simulink model "TB02_StageB_HBridge"  (R2025a)
settings: Solver=FixedStepDiscrete  StartTime=0  StopTime=TB.t_end  FixedStep=TB.dt  RelTol=1e-3
InitFcn:
  | % 모델과 같은 폴더의 초기화 스크립트를 실행해 P(설계 파라미터)와 TB(시험 조건)를 만든다.
  | run(fullfile(fileparts(get_param(bdroot, 'FileName')), 'TB02_init.m'));
values from neighbouring files (symbols this model uses):
  TB = struct()    [TB02_init.m]
libraries: fl_lib x20, nesl_utility x8
settings Model: Creator=hj000  LastModifiedBy=hj000
settings DataIOCC: SaveOutput=off  SignalLogging=off  SaveTime=off

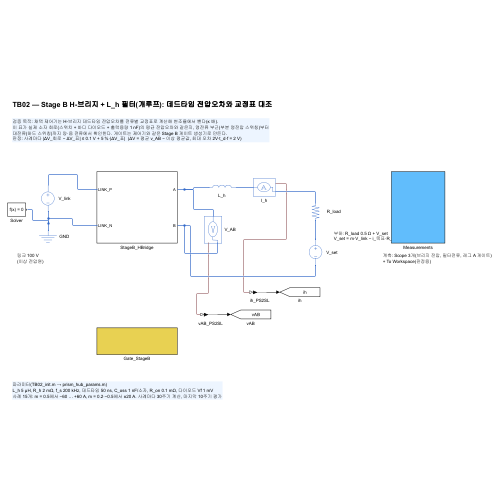
[thumbnail: Simulink's stored preview of the top-level diagram]
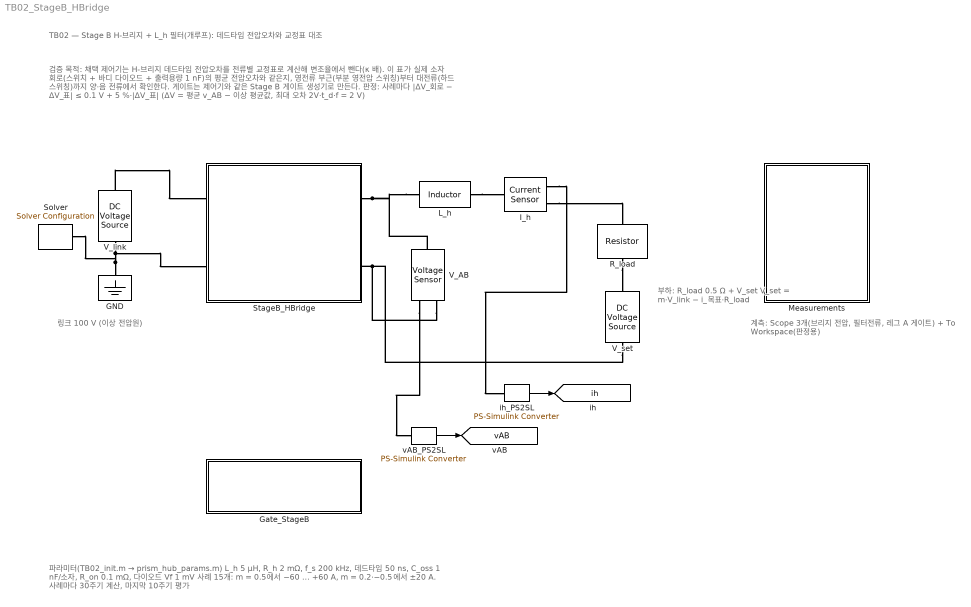
== system TB02_StageB_HBridge ==
  note: TB02 — Stage B H-브리지 + L_h 필터(개루프): 데드타임 전압오차와 교정표 대조
  note: 검증 목적: 채택 제어기는 H-브리지 데드타임 전압오차를 전류별 교정표로 계산해 변조율에서 뺀다(κ 배).
      | 이 표가 실제 소자 회로(스위치 + 바디 다이오드 + 출력용량 1 nF)의 평균 전압오차와 같은지, 영전류 부근(부분 영전압 스위칭)부터
      | 대전류(하드 스위칭)까지 양·음 전류에서 확인한다. 게이트는 제어기와 같은 Stage B 게이트 생성기로 만든다.
      | 판정: 사례마다 |ΔV_회로 − ΔV_표| ≤ 0.1 V + 5 %·|ΔV_표|  (ΔV = 평균 v_AB − 이상 평균값, 최대 오차 2V·t_d·f = 2 V)
  note: 링크 100 V
      | (이상 전압원)
  note: 부하: R_load 0.5 Ω + V_set
      | V_set = m·V_link − i_목표·R_load
  note: 계측: Scope 3개(브리지 전압, 필터전류, 레그 A 게이트)
      | + To Workspace(판정용)
  note: 파라미터(TB02_init.m → prism_hub_params.m)
      | L_h 5 µH, R_h 2 mΩ, f_s 200 kHz, 데드타임 50 ns, C_oss 1 nF/소자, R_on 0.1 mΩ, 다이오드 Vf 1 mV
      | 사례 15개: m = 0.5에서 −60 … +60 A, m = 0.2·−0.5에서 ±20 A. 사례마다 30주기 계산, 마지막 10주기 평가
  GND : fl_lib/Electrical/Electrical Elements/Electrical Reference
  Gate_StageB : Subsystem
  I_h : fl_lib/Electrical/Electrical Sensors/Current Sensor
  L_h : fl_lib/Electrical/Electrical Elements/Inductor  l=TB.B.Lh H  r=TB.B.Rh Ohm  g=1e-9 1/Ohm  i_specify=off  i_priority=None  i=0 A  i_nominal_specify=off  i_nominal_value=1  i_nominal_unit=A  v_specify=off  v_priority=None  v=0 V  v_nominal_specify=off  v_nominal_value=1  v_nominal_unit=V  i_L_specify=on  i_L_priority=High  i_L=TB.i0 A  i_L_nominal_specify=off  i_L_nominal_value=1  i_L_nominal_unit=A
  Measurements : Subsystem
  R_load : fl_lib/Electrical/Electrical Elements/Resistor  R=TB.Rload Ohm  i_specify=off  i_priority=None  i=0 A  i_nominal_specify=off  i_nominal_value=1  i_nominal_unit=A  v_specify=off  v_priority=None  v=0 V  v_nominal_specify=off  v_nominal_value=1  v_nominal_unit=V
  Solver : nesl_utility/Solver Configuration  PhysicalDomain=network_engine_domain  SubClassName=solver  LeftPortType=input  RightPortType=generic  Tones=[]  Harmonics=[]  SimulateNoise=off  Profile=off  UseLocalSampling=off  EnableSwitchedLinearOptims=on  FrequencyDomain=off  UseCCode=off  RelTol=0.001  AbsTol=0.001  MinStep=1e-09  ToWorkspace=off  RevertToSquareIcSolve=off  NumHomotopyIterations=100  PhasorMode=off  PhasorModeNumHarmonics=1  ConsistencySolver=NEWTON_XTOL_AFTER_FTOL  IndexReductionMethod=DerivativeReplacement  DoDC=off  ResidualTolerance=1e-9  ConsistencyTolSource=GLOBAL  ConsistencyAbsTol=0.001  ConsistencyRelTol=0.001  ConsistencyTolFactor=0.001  UseLocalSolver=on  LocalSolverChoice=NE_BACKWARD_EULER_ADVANCER  ResolveIndetEquations=on  FunctionEvalNumThread=1  LocalSolverSampleTime=TB.dt  DoFixedCost=off  MaxNonlinIter=3  MaxModeIter=2  ComputeImpulses=off  ImpulseIterations=2  LinearAlgebra=auto  LinearAlgebraNumThread=0  EquationFormulation=NE_TIME_EF  DelaysMemoryBudget=1024  AutomaticFiltering=on  FilteringTimeConstant=0.001  PartitionStorageMethod=AS_NEEDED  PartitionMemoryBudget=1024  PartitionMethod=ROBUST  MultibodyUseLocalSolver=off  MultibodyLocalSolverChoice=ODE1  MultibodyLocalSolverSampleTime=0.001
  StageB_HBridge : Subsystem
  V_AB : fl_lib/Electrical/Electrical Sensors/Voltage Sensor
  V_link : fl_lib/Electrical/Electrical Sources/DC Voltage Source  v0=TB.Vlink V
  V_set : fl_lib/Electrical/Electrical Sources/DC Voltage Source  v0=TB.Vset V
  ih_PS2SL : nesl_utility/PS-Simulink Converter  PhysicalDomain=network_engine_domain  SubClassName=ps_output  LeftPortType=input  RightPortType=output  PseudoPeriodic=off  Frequencies=[]  VectorFormat=inherit  Unit=inherit  AffineConversion=off
  vAB_PS2SL : nesl_utility/PS-Simulink Converter  PhysicalDomain=network_engine_domain  SubClassName=ps_output  LeftPortType=input  RightPortType=output  PseudoPeriodic=off  Frequencies=[]  VectorFormat=inherit  Unit=inherit  AffineConversion=off
  tag scope: ih=global, vAB=global
  wires:
  ih_PS2SL/1 -> [ih]
  vAB_PS2SL/1 -> [vAB]
  connections:
  GND/LConn1 -- Solver/RConn1 -- V_link/RConn1 -- StageB_HBridge/LConn2
  V_link/LConn1 -- StageB_HBridge/LConn1
  L_h/LConn1 -- StageB_HBridge/RConn1 -- V_AB/LConn1
  L_h/RConn1 -- I_h/LConn1
  I_h/RConn2 -- R_load/LConn1
  R_load/RConn1 -- V_set/LConn1
  StageB_HBridge/RConn2 -- V_set/RConn1 -- V_AB/RConn2
  I_h/RConn1 -- ih_PS2SL/LConn1
  V_AB/RConn1 -- vAB_PS2SL/LConn1

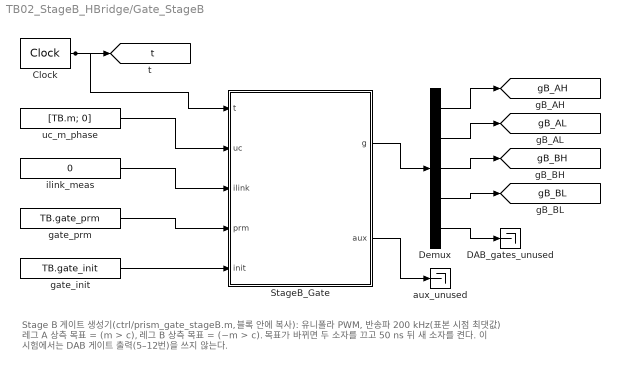
== system TB02_StageB_HBridge/Gate_StageB ==
  note: Stage B 게이트 생성기(ctrl/prism_gate_stageB.m, 블록 안에 복사): 유니폴라 PWM, 반송파 200 kHz(표본 시점 최댓값)
      | 레그 A 상측 목표 = (m > c), 레그 B 상측 목표 = (−m > c). 목표가 바뀌면 두 소자를 끄고 50 ns 뒤 새 소자를 켠다.
      | 이 시험에서는 DAB 게이트 출력(5–12번)을 쓰지 않는다.
  Clock : DigitalClock  SampleTime=TB.dt
  DAB_gates_unused : Terminator
  Demux : Demux  Outputs=[1 1 1 1 8]
  StageB_Gate : MATLAB Function  TreatAsAtomicUnit=on
  aux_unused : Terminator
  gate_init : Constant  Value=TB.gate_init
  gate_prm : Constant  Value=TB.gate_prm
  ilink_meas : Constant  Value=0
  uc_m_phase : Constant  Value=[TB.m; 0]
  tag scope: gB_AH=global, gB_AL=global, gB_BH=global, gB_BL=global, t=global
  wires:
  Clock/1 -> StageB_Gate/1(t), [t]
  uc_m_phase/1 -> StageB_Gate/2(uc)
  ilink_meas/1 -> StageB_Gate/3(ilink)
  gate_prm/1 -> StageB_Gate/4(prm)
  gate_init/1 -> StageB_Gate/5(init)
  StageB_Gate/1(g) -> Demux/1
  Demux/1 -> [gB_AH]
  Demux/2 -> [gB_AL]
  Demux/3 -> [gB_BH]
  Demux/4 -> [gB_BL]
  Demux/5 -> DAB_gates_unused/1
  StageB_Gate/2(aux) -> aux_unused/1

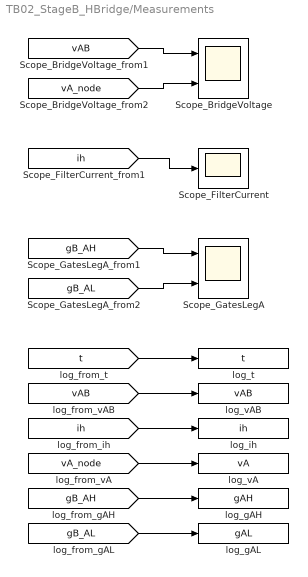
== system TB02_StageB_HBridge/Measurements ==
  Scope_BridgeVoltage : Scope  NumInputPorts=2
      settings: Title=Scope BridgeVoltage
  Scope_FilterCurrent : Scope
      settings: Title=Scope FilterCurrent
  Scope_GatesLegA : Scope  NumInputPorts=2
      settings: Title=Scope GatesLegA
  log_gAH : ToWorkspace  VariableName=gAH  SampleTime=-1
  log_gAL : ToWorkspace  VariableName=gAL  SampleTime=-1
  log_ih : ToWorkspace  VariableName=ih  SampleTime=-1
  log_t : ToWorkspace  VariableName=t  SampleTime=-1
  log_vA : ToWorkspace  VariableName=vA  SampleTime=-1
  log_vAB : ToWorkspace  VariableName=vAB  SampleTime=-1
  wires:
  [vAB] -> Scope_BridgeVoltage/1
  [vA_node] -> Scope_BridgeVoltage/2
  [ih] -> Scope_FilterCurrent/1
  [gB_AH] -> Scope_GatesLegA/1
  [gB_AL] -> Scope_GatesLegA/2
  [t] -> log_t/1
  [vAB] -> log_vAB/1
  [ih] -> log_ih/1
  [vA_node] -> log_vA/1
  [gB_AH] -> log_gAH/1
  [gB_AL] -> log_gAL/1

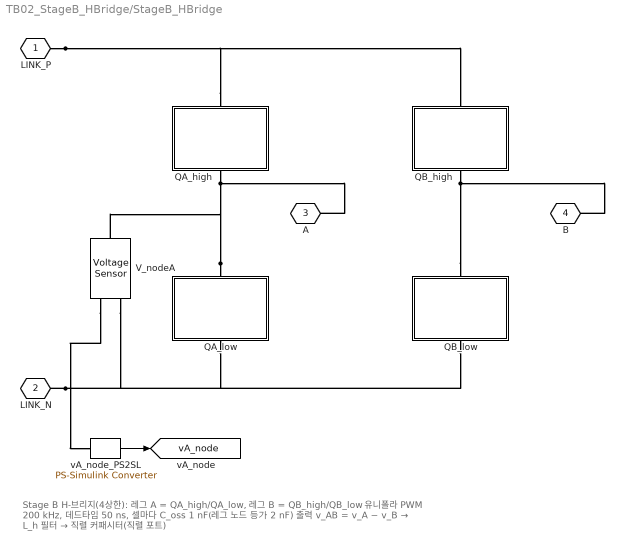
== system TB02_StageB_HBridge/StageB_HBridge ==
  note: Stage B H-브리지(4상한): 레그 A = QA_high/QA_low, 레그 B = QB_high/QB_low
      | 유니폴라 PWM 200 kHz, 데드타임 50 ns, 셀마다 C_oss 1 nF(레그 노드 등가 2 nF)
      | 출력 v_AB = v_A − v_B → L_h 필터 → 직렬 커패시터(직렬 포트)
  QA_high : Subsystem  mask(PRISM-Hub switch cell){Ron=TB.B.Ron, Goff=TB.B.Goff, Vf=TB.B.Vf, Rd=TB.B.Rd, Goffd=TB.B.Goffd, Coss=TB.B.Coss_h}
      mask prompts: Ron "도통 저항 R_on [Ohm]"; Goff "차단 컨덕턴스 G_off [S]"; Vf "다이오드 순방향 전압 Vf [V]"; Rd "다이오드 도통 저항 R_d [Ohm]"; Goffd "다이오드 차단 컨덕턴스 [S]"; Coss "출력용량 C_oss [F]"
      mask help: 전력 반도체 스위치 셀 QA_H. 게이트 태그 gB_AH.
      settings: AttributesFormatString=gate: gB_AH
      mask Display:
      | plot([0.50 0.50 ],[0.95 0.65 ],[0.50 0.74 ],[0.65 0.35 ],[0.50 0.50 ],[0.35 0.05 ]);
      | plot([0.50 0.20 0.20 ],[0.80 0.80 0.58 ],[0.20 0.20 0.50 ],[0.42 0.20 0.20 ]);
      | plot([0.20 0.10 0.30 0.20 ],[0.58 0.42 0.42 0.58 ],[0.10 0.30 ],[0.58 0.58 ]);
      | port_label('LConn',1,'D');
      | port_label('RConn',1,'S');
  QA_low : Subsystem  mask(PRISM-Hub switch cell){Ron=TB.B.Ron, Goff=TB.B.Goff, Vf=TB.B.Vf, Rd=TB.B.Rd, Goffd=TB.B.Goffd, Coss=TB.B.Coss_h}
      mask prompts: Ron "도통 저항 R_on [Ohm]"; Goff "차단 컨덕턴스 G_off [S]"; Vf "다이오드 순방향 전압 Vf [V]"; Rd "다이오드 도통 저항 R_d [Ohm]"; Goffd "다이오드 차단 컨덕턴스 [S]"; Coss "출력용량 C_oss [F]"
      mask help: 전력 반도체 스위치 셀 QA_L. 게이트 태그 gB_AL.
      settings: AttributesFormatString=gate: gB_AL
      mask Display:
      | plot([0.50 0.50 ],[0.95 0.65 ],[0.50 0.74 ],[0.65 0.35 ],[0.50 0.50 ],[0.35 0.05 ]);
      | plot([0.50 0.20 0.20 ],[0.80 0.80 0.58 ],[0.20 0.20 0.50 ],[0.42 0.20 0.20 ]);
      | plot([0.20 0.10 0.30 0.20 ],[0.58 0.42 0.42 0.58 ],[0.10 0.30 ],[0.58 0.58 ]);
      | port_label('LConn',1,'D');
      | port_label('RConn',1,'S');
  QB_high : Subsystem  mask(PRISM-Hub switch cell){Ron=TB.B.Ron, Goff=TB.B.Goff, Vf=TB.B.Vf, Rd=TB.B.Rd, Goffd=TB.B.Goffd, Coss=TB.B.Coss_h}
      mask prompts: Ron "도통 저항 R_on [Ohm]"; Goff "차단 컨덕턴스 G_off [S]"; Vf "다이오드 순방향 전압 Vf [V]"; Rd "다이오드 도통 저항 R_d [Ohm]"; Goffd "다이오드 차단 컨덕턴스 [S]"; Coss "출력용량 C_oss [F]"
      mask help: 전력 반도체 스위치 셀 QB_H. 게이트 태그 gB_BH.
      settings: AttributesFormatString=gate: gB_BH
      mask Display:
      | plot([0.50 0.50 ],[0.95 0.65 ],[0.50 0.74 ],[0.65 0.35 ],[0.50 0.50 ],[0.35 0.05 ]);
      | plot([0.50 0.20 0.20 ],[0.80 0.80 0.58 ],[0.20 0.20 0.50 ],[0.42 0.20 0.20 ]);
      | plot([0.20 0.10 0.30 0.20 ],[0.58 0.42 0.42 0.58 ],[0.10 0.30 ],[0.58 0.58 ]);
      | port_label('LConn',1,'D');
      | port_label('RConn',1,'S');
  QB_low : Subsystem  mask(PRISM-Hub switch cell){Ron=TB.B.Ron, Goff=TB.B.Goff, Vf=TB.B.Vf, Rd=TB.B.Rd, Goffd=TB.B.Goffd, Coss=TB.B.Coss_h}
      mask prompts: Ron "도통 저항 R_on [Ohm]"; Goff "차단 컨덕턴스 G_off [S]"; Vf "다이오드 순방향 전압 Vf [V]"; Rd "다이오드 도통 저항 R_d [Ohm]"; Goffd "다이오드 차단 컨덕턴스 [S]"; Coss "출력용량 C_oss [F]"
      mask help: 전력 반도체 스위치 셀 QB_L. 게이트 태그 gB_BL.
      settings: AttributesFormatString=gate: gB_BL
      mask Display:
      | plot([0.50 0.50 ],[0.95 0.65 ],[0.50 0.74 ],[0.65 0.35 ],[0.50 0.50 ],[0.35 0.05 ]);
      | plot([0.50 0.20 0.20 ],[0.80 0.80 0.58 ],[0.20 0.20 0.50 ],[0.42 0.20 0.20 ]);
      | plot([0.20 0.10 0.30 0.20 ],[0.58 0.42 0.42 0.58 ],[0.10 0.30 ],[0.58 0.58 ]);
      | port_label('LConn',1,'D');
      | port_label('RConn',1,'S');
  V_nodeA : fl_lib/Electrical/Electrical Sensors/Voltage Sensor
  vA_node_PS2SL : nesl_utility/PS-Simulink Converter  PhysicalDomain=network_engine_domain  SubClassName=ps_output  LeftPortType=input  RightPortType=output  PseudoPeriodic=off  Frequencies=[]  VectorFormat=inherit  Unit=inherit  AffineConversion=off
  LINK_P : PMIOPort  Side=Left
  LINK_N : PMIOPort  Port=2  Side=Left
  A : PMIOPort  Port=3  Side=Right
  B : PMIOPort  Port=4  Side=Right
  tag scope: vA_node=global
  wires:
  vA_node_PS2SL/1 -> [vA_node]
  connections:
  QA_high/LConn1 -- LINK_P/RConn1 -- QB_high/LConn1
  QA_high/RConn1 -- A/RConn1 -- QA_low/LConn1 -- V_nodeA/LConn1
  QB_low/LConn1 -- QB_high/RConn1 -- B/RConn1
  QA_low/RConn1 -- QB_low/RConn1 -- LINK_N/RConn1 -- V_nodeA/RConn2
  V_nodeA/RConn1 -- vA_node_PS2SL/LConn1

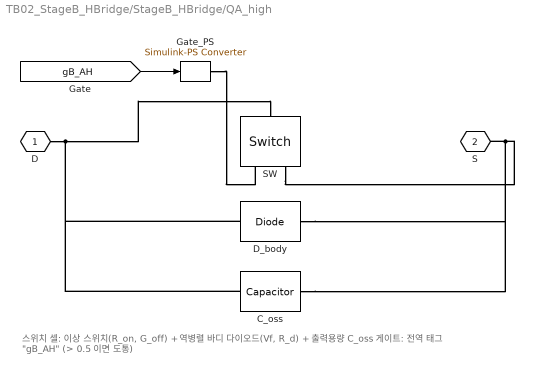
== system TB02_StageB_HBridge/StageB_HBridge/QA_high ==
  note: 스위치 셀: 이상 스위치(R_on, G_off) + 역병렬 바디 다이오드(Vf, R_d) + 출력용량 C_oss
      | 게이트: 전역 태그 "gB_AH" (> 0.5 이면 도통)
  C_oss : fl_lib/Electrical/Electrical Elements/Capacitor  c=Coss F  r=1e-6 Ohm  g=0 1/Ohm  i_specify=off  i_priority=None  i=0 A  i_nominal_specify=off  i_nominal_value=1  i_nominal_unit=A  v_specify=off  v_priority=None  v=0 V  v_nominal_specify=off  v_nominal_value=1  v_nominal_unit=V  vc_specify=off  vc_priority=High  vc=0 V  vc_nominal_specify=off  vc_nominal_value=1  vc_nominal_unit=V
  D_body : fl_lib/Electrical/Electrical Elements/Diode  Vf=Vf V  Ron=Rd Ohm  Goff=Goffd 1/Ohm  i_specify=off  i_priority=None  i=0 A  i_nominal_specify=off  i_nominal_value=1  i_nominal_unit=A  v_specify=off  v_priority=None  v=0 V  v_nominal_specify=off  v_nominal_value=1  v_nominal_unit=V
  Gate_PS : nesl_utility/Simulink-PS Converter  PhysicalDomain=network_engine_domain  SubClassName=ps_input  LeftPortType=input  RightPortType=output  PseudoPeriodic=off  Frequencies=[]  NoiseDistribution=none  NoiseParameters=[]  Unit=1  AffineConversion=off  FilteringAndDerivatives=zero  SimscapeFilterOrder=1  InputFilterTimeConstant=0.001  UdotUserProvided=0
  SW : fl_lib/Electrical/Electrical Elements/Switch  R_closed=Ron Ohm  G_open=Goff 1/Ohm  Threshold=0.5  i_specify=off  i_priority=None  i=0 A  i_nominal_specify=off  i_nominal_value=1  i_nominal_unit=A  v_specify=off  v_priority=None  v=0 V  v_nominal_specify=off  v_nominal_value=1  v_nominal_unit=V
  D : PMIOPort  Side=Left
  S : PMIOPort  Port=2  Side=Right
  wires:
  [gB_AH] -> Gate_PS/1
  connections:
  Gate_PS/RConn1 -- SW/RConn1
  SW/LConn1 -- D/RConn1 -- D_body/RConn1 -- C_oss/LConn1
  SW/RConn2 -- D_body/LConn1 -- S/RConn1 -- C_oss/RConn1

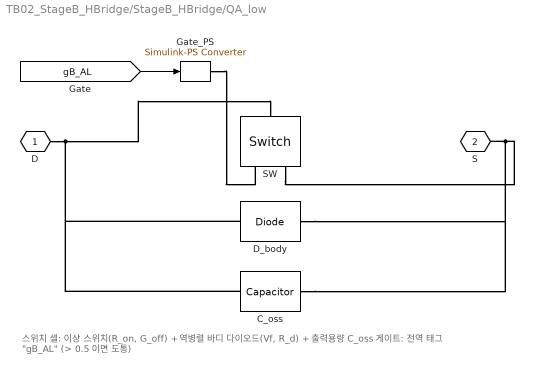
== system TB02_StageB_HBridge/StageB_HBridge/QA_low ==
  note: 스위치 셀: 이상 스위치(R_on, G_off) + 역병렬 바디 다이오드(Vf, R_d) + 출력용량 C_oss
      | 게이트: 전역 태그 "gB_AL" (> 0.5 이면 도통)
  C_oss : fl_lib/Electrical/Electrical Elements/Capacitor  c=Coss F  r=1e-6 Ohm  g=0 1/Ohm  i_specify=off  i_priority=None  i=0 A  i_nominal_specify=off  i_nominal_value=1  i_nominal_unit=A  v_specify=off  v_priority=None  v=0 V  v_nominal_specify=off  v_nominal_value=1  v_nominal_unit=V  vc_specify=off  vc_priority=High  vc=0 V  vc_nominal_specify=off  vc_nominal_value=1  vc_nominal_unit=V
  D_body : fl_lib/Electrical/Electrical Elements/Diode  Vf=Vf V  Ron=Rd Ohm  Goff=Goffd 1/Ohm  i_specify=off  i_priority=None  i=0 A  i_nominal_specify=off  i_nominal_value=1  i_nominal_unit=A  v_specify=off  v_priority=None  v=0 V  v_nominal_specify=off  v_nominal_value=1  v_nominal_unit=V
  Gate_PS : nesl_utility/Simulink-PS Converter  PhysicalDomain=network_engine_domain  SubClassName=ps_input  LeftPortType=input  RightPortType=output  PseudoPeriodic=off  Frequencies=[]  NoiseDistribution=none  NoiseParameters=[]  Unit=1  AffineConversion=off  FilteringAndDerivatives=zero  SimscapeFilterOrder=1  InputFilterTimeConstant=0.001  UdotUserProvided=0
  SW : fl_lib/Electrical/Electrical Elements/Switch  R_closed=Ron Ohm  G_open=Goff 1/Ohm  Threshold=0.5  i_specify=off  i_priority=None  i=0 A  i_nominal_specify=off  i_nominal_value=1  i_nominal_unit=A  v_specify=off  v_priority=None  v=0 V  v_nominal_specify=off  v_nominal_value=1  v_nominal_unit=V
  D : PMIOPort  Side=Left
  S : PMIOPort  Port=2  Side=Right
  wires:
  [gB_AL] -> Gate_PS/1
  connections:
  Gate_PS/RConn1 -- SW/RConn1
  SW/LConn1 -- D/RConn1 -- D_body/RConn1 -- C_oss/LConn1
  SW/RConn2 -- D_body/LConn1 -- S/RConn1 -- C_oss/RConn1

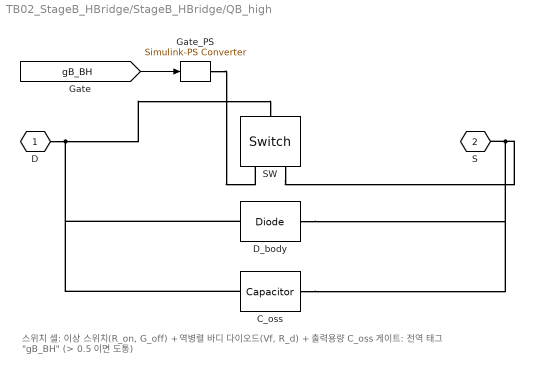
== system TB02_StageB_HBridge/StageB_HBridge/QB_high ==
  note: 스위치 셀: 이상 스위치(R_on, G_off) + 역병렬 바디 다이오드(Vf, R_d) + 출력용량 C_oss
      | 게이트: 전역 태그 "gB_BH" (> 0.5 이면 도통)
  C_oss : fl_lib/Electrical/Electrical Elements/Capacitor  c=Coss F  r=1e-6 Ohm  g=0 1/Ohm  i_specify=off  i_priority=None  i=0 A  i_nominal_specify=off  i_nominal_value=1  i_nominal_unit=A  v_specify=off  v_priority=None  v=0 V  v_nominal_specify=off  v_nominal_value=1  v_nominal_unit=V  vc_specify=off  vc_priority=High  vc=0 V  vc_nominal_specify=off  vc_nominal_value=1  vc_nominal_unit=V
  D_body : fl_lib/Electrical/Electrical Elements/Diode  Vf=Vf V  Ron=Rd Ohm  Goff=Goffd 1/Ohm  i_specify=off  i_priority=None  i=0 A  i_nominal_specify=off  i_nominal_value=1  i_nominal_unit=A  v_specify=off  v_priority=None  v=0 V  v_nominal_specify=off  v_nominal_value=1  v_nominal_unit=V
  Gate_PS : nesl_utility/Simulink-PS Converter  PhysicalDomain=network_engine_domain  SubClassName=ps_input  LeftPortType=input  RightPortType=output  PseudoPeriodic=off  Frequencies=[]  NoiseDistribution=none  NoiseParameters=[]  Unit=1  AffineConversion=off  FilteringAndDerivatives=zero  SimscapeFilterOrder=1  InputFilterTimeConstant=0.001  UdotUserProvided=0
  SW : fl_lib/Electrical/Electrical Elements/Switch  R_closed=Ron Ohm  G_open=Goff 1/Ohm  Threshold=0.5  i_specify=off  i_priority=None  i=0 A  i_nominal_specify=off  i_nominal_value=1  i_nominal_unit=A  v_specify=off  v_priority=None  v=0 V  v_nominal_specify=off  v_nominal_value=1  v_nominal_unit=V
  D : PMIOPort  Side=Left
  S : PMIOPort  Port=2  Side=Right
  wires:
  [gB_BH] -> Gate_PS/1
  connections:
  Gate_PS/RConn1 -- SW/RConn1
  SW/LConn1 -- D/RConn1 -- D_body/RConn1 -- C_oss/LConn1
  SW/RConn2 -- D_body/LConn1 -- S/RConn1 -- C_oss/RConn1

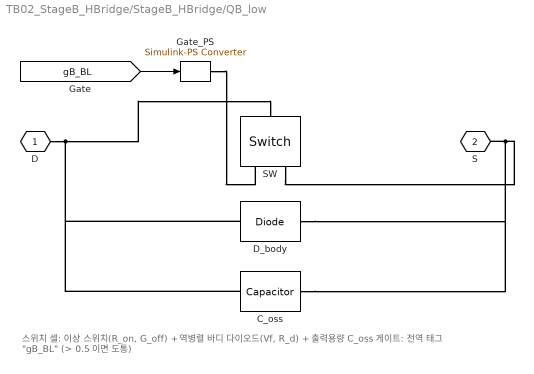
== system TB02_StageB_HBridge/StageB_HBridge/QB_low ==
  note: 스위치 셀: 이상 스위치(R_on, G_off) + 역병렬 바디 다이오드(Vf, R_d) + 출력용량 C_oss
      | 게이트: 전역 태그 "gB_BL" (> 0.5 이면 도통)
  C_oss : fl_lib/Electrical/Electrical Elements/Capacitor  c=Coss F  r=1e-6 Ohm  g=0 1/Ohm  i_specify=off  i_priority=None  i=0 A  i_nominal_specify=off  i_nominal_value=1  i_nominal_unit=A  v_specify=off  v_priority=None  v=0 V  v_nominal_specify=off  v_nominal_value=1  v_nominal_unit=V  vc_specify=off  vc_priority=High  vc=0 V  vc_nominal_specify=off  vc_nominal_value=1  vc_nominal_unit=V
  D_body : fl_lib/Electrical/Electrical Elements/Diode  Vf=Vf V  Ron=Rd Ohm  Goff=Goffd 1/Ohm  i_specify=off  i_priority=None  i=0 A  i_nominal_specify=off  i_nominal_value=1  i_nominal_unit=A  v_specify=off  v_priority=None  v=0 V  v_nominal_specify=off  v_nominal_value=1  v_nominal_unit=V
  Gate_PS : nesl_utility/Simulink-PS Converter  PhysicalDomain=network_engine_domain  SubClassName=ps_input  LeftPortType=input  RightPortType=output  PseudoPeriodic=off  Frequencies=[]  NoiseDistribution=none  NoiseParameters=[]  Unit=1  AffineConversion=off  FilteringAndDerivatives=zero  SimscapeFilterOrder=1  InputFilterTimeConstant=0.001  UdotUserProvided=0
  SW : fl_lib/Electrical/Electrical Elements/Switch  R_closed=Ron Ohm  G_open=Goff 1/Ohm  Threshold=0.5  i_specify=off  i_priority=None  i=0 A  i_nominal_specify=off  i_nominal_value=1  i_nominal_unit=A  v_specify=off  v_priority=None  v=0 V  v_nominal_specify=off  v_nominal_value=1  v_nominal_unit=V
  D : PMIOPort  Side=Left
  S : PMIOPort  Port=2  Side=Right
  wires:
  [gB_BL] -> Gate_PS/1
  connections:
  Gate_PS/RConn1 -- SW/RConn1
  SW/LConn1 -- D/RConn1 -- D_body/RConn1 -- C_oss/LConn1
  SW/RConn2 -- D_body/LConn1 -- S/RConn1 -- C_oss/RConn1

== matlab function TB02_StageB_HBridge/Gate_StageB/StageB_Gate ==
  data: t input; g output; uc input; ilink input; prm input; init input; aux output
function [g, aux] = prism_gate_stageB(t, uc, ilink, prm, init)
%#codegen
%PRISM_GATE_STAGEB  Stage B 게이트 생성기(적분 간격 dt = 5 ns마다 실행).
%
%  H-브리지 : 유니폴라 PWM. 삼각 반송파 c(t)는 제어주기 시작(표본 시점)에서 +1, 반주기에서 −1.
%             레그 A 상측 목표 = (m > c), 레그 B 상측 목표 = (−m > c). 목표가 바뀌면 두 소자를 데드타임 동안
%             끄고(출력용량 충방전·다이오드 도통은 회로가 정함) 새 소자를 켠다.
%  DAB      : 50 % 구형파 두 풀브리지, 단일 위상천이. 에지는 반송파 반주기 중심 c_j에 대칭(1차 c_j − δ/2,
%             2차 c_j + δ/2, δ = φ·T/2π)으로 놓고, 지령은 도착 후 첫 반주기 중심에서 반영한다.
%             전이 반주기의 위상차를 이전·새 위상의 평균으로 두는 갱신(A ← −A + 2Δ, Δ = (A + δ_new)/2)으로
%             위상이 바뀔 때 변압기 직류 편류가 생기지 않게 한다(검증 코드와 같은 알고리즘).
%             에지 시각은 dt 격자에 반올림하고, 실제 실행 시각으로 다음 반주기의 A를 계산한다.
%  링크전류 : DAB 2차 브리지가 링크로 보내는 직류전류를 제어주기마다 평균해 다음 표본에 넘긴다.
%
%  입력  t      시뮬레이션 시각(Digital Clock, dt 간격)
%        uc     [PWM 비교값; DAB 유효 위상 rad]  (제어기 출력, 전달지연 뒤)
%        ilink  DAB 2차 브리지 → 링크 직류전류 [A](순시)
%        prm    [dt Np td_h(간격 수) td_d(간격 수) T]
%        init   [PWM 비교값 초기값, 위상 초기값, 링크전류 초기값]
%  출력  g      [A상측 A하측 B상측 B하측 | P1 P2 P3 P4 | S1 S2 S3 S4]  (1 = 켬)
%               DAB 브리지: 상태 +1 → 1·4번 켬, −1 → 2·3번 켬(1·2번이 레그 1, 3·4번이 레그 2, 홀수 = 상측)
%        aux    [링크전류 주기 평균; 그 주기 두 반주기 중심의 위상 φ_c0, φ_c1; 반송파; 1차 상태; 2차 상태]

persistent started kA kB tgtA tgtB A ph_tgt p_t s_t p_h s_h p_j s_j p_state s_state p_te s_te ...
           acc il_avg phc0 phc1 lat0 lat1
dt = prm(1); Np = prm(2); ndh = prm(3); ndd = prm(4); T = prm(5);
Nh = round(Np/2);
k  = round(t/dt);                     % 적분 간격 번호(0부터)
t0 = k*dt;

if isempty(started)
    started = 1;
    m0 = init(1); ph0 = init(2);
    c0 = 1;                            % k = 0의 반송파
    tgtA = double(m0 > c0); tgtB = double(-m0 > c0);
    kA = -1e9; kB = -1e9;              % 데드타임 없이 시작
    ph_tgt = ph0;
    d0 = ph0/(2*pi)*T;
    A = d0;
    p_t = [1e30 1e30]; s_t = [1e30 1e30]; p_h = [0 0]; s_h = [0 0];
    p_te = -1; s_te = -1;
    if d0 > 0
        p_j = 1; p_h(1) = -d0/2; p_state = 1;  s_j = 0; s_state = -1;
    elseif d0 < 0
        s_j = 1; s_h(1) = d0/2;  s_state = 1;  p_j = 0; p_state = -1;
    else
        p_j = 0; s_j = 0; p_state = -1; s_state = -1;
    end
    acc = 0; il_avg = init(3); phc0 = ph0; phc1 = ph0; lat0 = ph0; lat1 = ph0;
end

m = uc(1);
ph_tgt = uc(2);

% ---------------- H-브리지 유니폴라 PWM -------------------------------------------------
kin = mod(k, Np);
c = 4*abs(kin/Np - 0.5) - 1;
nA = double(m > c); nB = double(-m > c);
if nA ~= tgtA, tgtA = nA; kA = k; end
if nB ~= tgtB, tgtB = nB; kB = k; end
okA = (k - kA) >= ndh; okB = (k - kB) >= ndh;
gA_hi = double(okA && tgtA == 1); gA_lo = double(okA && tgtA == 0);
gB_hi = double(okB && tgtB == 1); gB_lo = double(okB && tgtB == 0);

% ---------------- DAB 위상 갱신(반주기 중심) --------------------------------------------
if mod(k, Nh) == 0
    j = k/Nh; cj = t0;
    if j >= 1
        jm = mod(j - 1, 2) + 1;
        A = -A + 2*(s_h(jm) - p_h(jm));
    end
    dtg = ph_tgt/(2*pi)*T;
    D = 0.5*(A + dtg);
    jj = mod(j, 2) + 1;
    p_done = p_j > j; s_done = s_j > j;
    if p_done && ~s_done
        s_t(jj) = max(cj, p_h(jj) + D);
    elseif s_done && ~p_done
        p_t(jj) = max(cj, s_h(jj) - D);
    elseif ~p_done && ~s_done
        if D >= 0
            p_t(jj) = cj; s_t(jj) = cj + D;
        else
            s_t(jj) = cj; p_t(jj) = cj - D;
        end
    end
    if p_done, tpj = p_h(jj); else, tpj = p_t(jj); end
    if s_done, tsj = s_h(jj); else, tsj = s_t(jj); end
    D1 = 0.5*(-A + 2*(tsj - tpj) + dtg);
    cn = (j + 1)*Nh*dt;
    p_t(3 - jj) = cn - D1/2; s_t(3 - jj) = cn + D1/2;
    if mod(j, 2) == 0, phc0 = ph_tgt; else, phc1 = ph_tgt; end
end
% ---------------- DAB 에지 실행(가장 가까운 간격에 반올림) ------------------------------
sp = mod(p_j, 2) + 1;
if p_t(sp) < t0 + 0.5*dt
    if mod(p_j, 2) == 0, p_state = 1; else, p_state = -1; end
    p_te = t0; p_h(sp) = t0; p_t(sp) = 1e30; p_j = p_j + 1;
end
ss = mod(s_j, 2) + 1;
if s_t(ss) < t0 + 0.5*dt
    if mod(s_j, 2) == 0, s_state = 1; else, s_state = -1; end
    s_te = t0; s_h(ss) = t0; s_t(ss) = 1e30; s_j = s_j + 1;
end
p_ok = (t0 - p_te) >= ndd*dt - 0.5*dt;
s_ok = (t0 - s_te) >= ndd*dt - 0.5*dt;
gP = [0 0 0 0]; gS = [0 0 0 0];
if p_ok
    if p_state > 0, gP = [1 0 0 1]; else, gP = [0 1 1 0]; end
end
if s_ok
    if s_state > 0, gS = [1 0 0 1]; else, gS = [0 1 1 0]; end
end

% ---------------- 링크전류 주기 평균(표본 직전 간격에서 확정) -------------------------
acc = acc + ilink;
if kin == Np - 1
    il_avg = acc/Np; acc = 0;
    lat0 = phc0; lat1 = phc1;
end

g = [gA_hi gA_lo gB_hi gB_lo gP gS]';
aux = [il_avg; lat0; lat1; c; p_state; s_state];
end
